simulink library "Lib_Piccolo"  (R2018b)
settings: Solver=VariableStepAuto  StartTime=0.0  StopTime=10.0  RelTol=1e-3
values from neighbouring files (symbols this model uses):
  AccelErrInt2Brakes = 0.15    [SimulationControlConfig16P.m]    (also in SimulationControlConfig16P_LEGACY.m; SimulationControlConfigTAILLESS.m = 0.2; SimulationControlConfigUTAIL.m = 0.2)
  AileronMax = 25    [SimulationControlConfig16P.m]    (also in SimulationControlConfig16P_LEGACY.m; SimulationControlConfigTAILLESS.m; SimulationControlConfigUTAIL.m)
  AileronPower = 0.00268    [SimulationControlConfig16P.m]    (also in SimulationControlConfig16P_LEGACY.m; SimulationControlConfigTAILLESS.m; SimulationControlConfigUTAIL.m)
  AileronSurfaceMax = 45    [SimulationControlConfig16P.m]    (also in SimulationControlConfig16P_LEGACY.m)
  AileronTrim = 0    [SimulationControlConfig16P.m]    (also in SimulationControlConfig16P_LEGACY.m; SimulationControlConfigTAILLESS.m; SimulationControlConfigUTAIL.m)
  Alt = 1000 + TerrainHeight    [SimulationStateConfig.m]
  AltCruise_m = testPlans(testIndx).terrainElevation * 0.3048 + 200    [SimulationControlConfig16P.m]    (also in SimulationControlConfigTAILLESS.m = 1083; SimulationControlConfigUTAIL.m = testPlans(testIndx).terrainElevation * 0.3048 + 152)
  AltitudeRate2PitchCmdIntegratorInit = 0.1    [SimulationControlPre.m]
  AltMax = 10000    [SimulationControlConfig16P.m]    (also in SimulationControlConfig16P_LEGACY.m; SimulationControlConfigTAILLESS.m; SimulationControlConfigUTAIL.m)
  AltMaxAccel = 1.25    [SimulationControlConfig16P.m]    (also in SimulationControlConfig16P_LEGACY.m = 0.9; SimulationControlConfigTAILLESS.m = 1.7; SimulationControlConfigUTAIL.m = 2)
  AltMin = 0    [SimulationControlConfig16P.m]    (also in SimulationControlConfig16P_LEGACY.m; SimulationControlConfigTAILLESS.m; SimulationControlConfigUTAIL.m)
  AltRateCmd2Pitch = 0.50    (= 0.5)    [SimulationControlConfig16P.m]    (also in SimulationControlConfig16P_LEGACY.m = 0.6; SimulationControlConfigTAILLESS.m = 0.2; SimulationControlConfigUTAIL.m = 0.3)
  AltRateError2Pitch = 0.40    (= 0.4)    [SimulationControlConfig16P.m]    (also in SimulationControlConfig16P_LEGACY.m; SimulationControlConfigTAILLESS.m = 0.55; SimulationControlConfigUTAIL.m = 0.55)
  AltRateErrorInt2Pitch = 0.50    (= 0.5)    [SimulationControlConfig16P.m]    (also in SimulationControlConfig16P_LEGACY.m = 0.45; SimulationControlConfigTAILLESS.m; SimulationControlConfigUTAIL.m = 0.75)
  AltRateLpfCutOff = 3    [SimulationControlConfig16P.m]    (also in SimulationControlConfig16P_LEGACY.m; SimulationControlConfigTAILLESS.m = 2; SimulationControlConfigUTAIL.m = 2)
  AutoNosegear2Rudder = 26    [SimulationControlConfig16P.m]    (also in SimulationControlConfig16P_LEGACY.m; SimulationControlConfigTAILLESS.m = 25.2; SimulationControlConfigUTAIL.m = 14)
  b = 5.54    [SimulationControlConfig16P.m]    (also in SimulationControlConfig16P_LEGACY.m; SimulationControlConfigTAILLESS.m = 2.37; SimulationControlConfigUTAIL.m = 2.37)
  Bank2AileronIntegratorInit = 0    [SimulationControlPre.m]
  BankMax_User = BankMax_User/180*pi    (= 0.523598775598)    [SimulationControlConfig16P.m]    (also in SimulationControlConfig16P_LEGACY.m; SimulationControlConfigTAILLESS.m = 0.610865238198; SimulationControlConfigUTAIL.m = 0.628318530718)
  baseLegFlaps = 20    [SimulationControlConfig16P.m]    (also in SimulationControlConfig16P_LEGACY.m = 0; SimulationControlConfigTAILLESS.m = 15; SimulationControlConfigUTAIL.m = 10)
  C = GeneticOpt.C    [SimulationCostFunction.m]
  c = Sw/b    (= 0.841696750903)    [SimulationControlConfig16P.m]    (also in SimulationControlConfig16P_LEGACY.m; SimulationControlConfigTAILLESS.m = 0.354008438819; SimulationControlConfigUTAIL.m = 0.354008438819)
  cell2WheelFactorMG = 5.98    [SimulationSensorConfig16P_LEGACY.m]
  cell2WheelFactorNG = 1    [SimulationSensorConfig16P_LEGACY.m]
  cellSatMaxMG = 15000    [SimulationSensorConfig16P.m]    (also in SimulationSensorConfig16P_LEGACY.m; SimulationSensorConfigTAILLESS7P.m; SimulationSensorConfigUTAIL7P.m)
  cellSatMaxNG = 1000    [SimulationSensorConfig16P.m]    (also in SimulationSensorConfig16P_LEGACY.m; SimulationSensorConfigTAILLESS7P.m; SimulationSensorConfigUTAIL7P.m)
  cellSatMinMG = -15000    [SimulationSensorConfig16P.m]    (also in SimulationSensorConfig16P_LEGACY.m; SimulationSensorConfigTAILLESS7P.m; SimulationSensorConfigUTAIL7P.m)
  cellSatMinNG = -1000    [SimulationSensorConfig16P.m]    (also in SimulationSensorConfig16P_LEGACY.m; SimulationSensorConfigTAILLESS7P.m; SimulationSensorConfigUTAIL7P.m)
  CL_Limit = CL_Max    (= 0.54)    [SimulationControlConfig16P.m]    (also in SimulationControlConfig16P_LEGACY.m; SimulationControlConfigTAILLESS.m; SimulationControlConfigUTAIL.m = 0.53)
  CL_Max = 0.54    [SimulationControlConfig16P.m]    (also in SimulationControlConfig16P_LEGACY.m; SimulationControlConfigTAILLESS.m; SimulationControlConfigUTAIL.m = 0.53)
  CL_Max_Nom = 0.465    [SimulationControlConfig16P.m]    (also in SimulationControlConfig16P_LEGACY.m; SimulationControlConfigTAILLESS.m = 0.39; SimulationControlConfigUTAIL.m)
  CL_Min = 0    [SimulationControlConfig16P.m]    (also in SimulationControlConfig16P_LEGACY.m; SimulationControlConfigTAILLESS.m; SimulationControlConfigUTAIL.m)
  ClimbMaxFraction = 0.35    [SimulationControlConfig16P.m]    (also in SimulationControlConfig16P_LEGACY.m = 0.24; SimulationControlConfigTAILLESS.m = 0.19; SimulationControlConfigUTAIL.m = 0.21)
  ClimboutMaxBank = 7.0    (= 7)    [SimulationControlConfig16P.m]    (also in SimulationControlConfig16P_LEGACY.m; SimulationControlConfigTAILLESS.m = 5; SimulationControlConfigUTAIL.m)
  ClimboutTimer = 7.0    (= 7)    [SimulationControlConfig16P.m]    (also in SimulationControlConfig16P_LEGACY.m; SimulationControlConfigTAILLESS.m; SimulationControlConfigUTAIL.m)
  dCl_per_dFlap = 0.005581818    [SimulationControlConfig16P.m]    (also in SimulationControlConfig16P_LEGACY.m = 0; SimulationControlConfigTAILLESS.m = 0; SimulationControlConfigUTAIL.m = 0)
  DecelerationCmd = 3.1    [SimulationControlConfig16P.m]    (also in SimulationControlConfig16P_LEGACY.m; SimulationControlConfigTAILLESS.m = 0.1; SimulationControlConfigUTAIL.m = 0.1)
  DeRotateLogicEndTimer = abs((NoseDownLimit_Deg-1)/DeRotateRamp_Dps)    [SimulationControlConfig16P.m]    (also in SimulationControlConfig16P_LEGACY.m; SimulationControlConfigTAILLESS.m; SimulationControlConfigUTAIL.m)
  DeRotateLogicHoldNoseUpTimer = 0.1    [SimulationControlConfig16P.m]    (also in SimulationControlConfig16P_LEGACY.m; SimulationControlConfigTAILLESS.m; SimulationControlConfigUTAIL.m)
  DeRotateLogicTimerTimeout = 2    [SimulationControlConfig16P.m]    (also in SimulationControlConfig16P_LEGACY.m; SimulationControlConfigTAILLESS.m; SimulationControlConfigUTAIL.m)
  DeRotateLowerCmdSaturation = 0    [SimulationControlConfig16P.m]    (also in SimulationControlConfig16P_LEGACY.m; SimulationControlConfigTAILLESS.m; SimulationControlConfigUTAIL.m)
  DeRotateRamp_Dps = 3    [SimulationControlConfig16P.m]    (also in SimulationControlConfig16P_LEGACY.m; SimulationControlConfigTAILLESS.m = 8; SimulationControlConfigUTAIL.m = 8)
  DeRotateUpperCmdSaturation = 7    [SimulationControlConfig16P.m]    (also in SimulationControlConfig16P_LEGACY.m; SimulationControlConfigTAILLESS.m; SimulationControlConfigUTAIL.m)
  DescentMaxFraction = 0.22    [SimulationControlConfig16P.m]    (also in SimulationControlConfig16P_LEGACY.m = 0.2; SimulationControlConfigTAILLESS.m = 0.17; SimulationControlConfigUTAIL.m = 0.17)
  DesktopSimTerrainOffset_m = 0.406    [SimulationAircraftConfig.m]
  downwindFlaps = 0    [SimulationControlConfig16P.m]    (also in SimulationControlConfig16P_LEGACY.m; SimulationControlConfigTAILLESS.m; SimulationControlConfigUTAIL.m)
  DP_init = 0.5*1.225*V_init^2    [SimulationControlConfig16P.m]    (also in SimulationControlConfig16P_LEGACY.m; SimulationControlConfigTAILLESS.m; SimulationControlConfigUTAIL.m)
  dscNoiseMG = 1    [SimulationSensorConfig16P_LEGACY.m]
  dscNoiseNG = 0.25    [SimulationSensorConfig16P_LEGACY.m]
  DSCnumBits = 24    [SimulationSensorConfig16P.m]    (also in SimulationSensorConfig16P_LEGACY.m; SimulationSensorConfigTAILLESS7P.m; SimulationSensorConfigUTAIL7P.m)
  DSCRangeMaxMG = 15000    [SimulationSensorConfig16P.m]    (also in SimulationSensorConfig16P_LEGACY.m; SimulationSensorConfigTAILLESS7P.m; SimulationSensorConfigUTAIL7P.m)
  DSCRangeMaxNG = 1000    [SimulationSensorConfig16P.m]    (also in SimulationSensorConfig16P_LEGACY.m; SimulationSensorConfigTAILLESS7P.m; SimulationSensorConfigUTAIL7P.m)
  DSCRangeMinMG = -15000    [SimulationSensorConfig16P.m]    (also in SimulationSensorConfig16P_LEGACY.m; SimulationSensorConfigTAILLESS7P.m; SimulationSensorConfigUTAIL7P.m)
  DSCRangeMinNG = -1000    [SimulationSensorConfig16P.m]    (also in SimulationSensorConfig16P_LEGACY.m; SimulationSensorConfigTAILLESS7P.m; SimulationSensorConfigUTAIL7P.m)
  dt = DLLSim.dt    [SimulationTimeStep.m]    (also in SimulationTrim.m = 0.02)
  EarlyTouchdownThreshold = 3.0    (= 3)    [SimulationControlConfig16P.m]    (also in SimulationControlConfig16P_LEGACY.m; SimulationControlConfigTAILLESS.m = 2.2; SimulationControlConfigUTAIL.m = 2.5)
  ElevatorDeflectionRate = 15    [SimulationControlConfig16P.m]    (also in SimulationControlConfig16P_LEGACY.m = 12; SimulationControlConfigTAILLESS.m = 10; SimulationControlConfigUTAIL.m = 12)
  ElevatorMax = 25    [SimulationControlConfig16P.m]    (also in SimulationControlConfig16P_LEGACY.m; SimulationControlConfigTAILLESS.m; SimulationControlConfigUTAIL.m)
  ElevatorPower = -0.002209    [SimulationControlConfig16P.m]    (also in SimulationControlConfig16P_LEGACY.m; SimulationControlConfigTAILLESS.m = -0.002956; SimulationControlConfigUTAIL.m = -0.00205983)
  ElevatorTrim = -3.5    [SimulationControlConfig16P.m]    (also in SimulationControlConfig16P_LEGACY.m; SimulationControlConfigTAILLESS.m = -6; SimulationControlConfigUTAIL.m = -8)
  elevonBias = 0    [SimulationControlConfig16P.m]    (also in SimulationControlConfig16P_LEGACY.m; SimulationControlConfigTAILLESS.m; SimulationControlConfigUTAIL.m)
  Enable_TAS_Protection = 0    [SimulationControlConfig16P.m]    (also in SimulationControlConfig16P_LEGACY.m; SimulationControlConfigTAILLESS.m; SimulationControlConfigUTAIL.m)
  EnableCrossTrackAbort = 1    [SimulationControlConfig16P.m]    (also in SimulationControlConfigTAILLESS.m; SimulationControlConfigUTAIL.m)
  EnergyBandwidth = 0.02    [SimulationControlConfig16P.m]    (also in SimulationControlConfig16P_LEGACY.m; SimulationControlConfigTAILLESS.m = 0.06; SimulationControlConfigUTAIL.m = 0.06)
  EngineLhFuelCut = 0    [SimulationAircraftConfig.m]
  EngineRhFuelCut = 0    [SimulationAircraftConfig.m]
  FastThrottleRate = 0.075    [SimulationControlConfig16P.m]    (also in SimulationControlConfig16P_LEGACY.m = 0.05; SimulationControlConfigTAILLESS.m = 0.1; SimulationControlConfigUTAIL.m = 0.1)
  FilterWarmUpTime = 2    [SimulationSensorConfig16P.m]    (also in SimulationSensorConfig16P_LEGACY.m; SimulationSensorConfigTAILLESS7P.m; SimulationSensorConfigUTAIL7P.m)
  finalApproachFlaps = 20    [SimulationControlConfig16P.m]    (also in SimulationControlConfig16P_LEGACY.m = 0; SimulationControlConfigTAILLESS.m = 22; SimulationControlConfigUTAIL.m = 10)
  FinalDescentSlope_Deg = testPlans(testIndx).descentSlope    [SimulationControlConfig16P.m]    (also in SimulationControlConfig16P_LEGACY.m; SimulationControlConfigTAILLESS.m; SimulationControlConfigUTAIL.m)
  flapMax = 0    [SimulationControlConfig16P.m]    (also in SimulationControlConfig16P_LEGACY.m; SimulationControlConfigTAILLESS.m; SimulationControlConfigUTAIL.m)
  flapRate = 7.5    [SimulationControlConfig16P.m]    (also in SimulationControlConfig16P_LEGACY.m; SimulationControlConfigTAILLESS.m = 6.6; SimulationControlConfigUTAIL.m)
  FlareHeight = 5    [SimulationControlConfig16P.m]    (also in SimulationControlConfig16P_LEGACY.m = 4.8; SimulationControlConfigTAILLESS.m = 2.5; SimulationControlConfigUTAIL.m = 2)
  FlareVerticalRate_mps = -0.4    [SimulationControlConfig16P.m]    (also in SimulationControlConfig16P_LEGACY.m = -0.5; SimulationControlConfigTAILLESS.m = -0.15; SimulationControlConfigUTAIL.m = -0.15)
  Fp_Aileron = 0.55*2*pi*RollRateLpfCutoff*dt    [SimulationControlConfig16P.m]    (also in SimulationControlConfig16P_LEGACY.m; SimulationControlConfigTAILLESS.m; SimulationControlConfigUTAIL.m)
  Fp_Alt = 0.55*AltBandwidth    (= 0.099)    [SimulationControlConfig16P.m]    (also in SimulationControlConfig16P_LEGACY.m; SimulationControlConfigTAILLESS.m = 0.587477826221; SimulationControlConfigUTAIL.m = 0.69115038379)
  Fp_AltRate = 0.55*2*pi*AltRateLpfCutOff*dt    [SimulationControlConfig16P.m]    (also in SimulationControlConfig16P_LEGACY.m; SimulationControlConfigTAILLESS.m; SimulationControlConfigUTAIL.m)
  Fp_Elevator = 0.55*2*pi*PitchRateLpfCutoff*dt    [SimulationControlConfig16P.m]    (also in SimulationControlConfig16P_LEGACY.m; SimulationControlConfigTAILLESS.m; SimulationControlConfigUTAIL.m)
  Fp_Energy = 0.55*2*pi*EnergyBandwidth    (= 0.069115038379)    [SimulationControlConfig16P.m]    (also in SimulationControlConfig16P_LEGACY.m; SimulationControlConfigTAILLESS.m = 0.207345115137; SimulationControlConfigUTAIL.m = 0.207345115137)
  Fp_Energy2 = 0.55*2*pi*EnergyBandwidth*dt    [SimulationControlConfig16P.m]    (also in SimulationControlConfig16P_LEGACY.m; SimulationControlConfigTAILLESS.m; SimulationControlConfigUTAIL.m)
  Fp_Pitch = 0.55*2*pi*PitchBandwidth    (= 2.76460153516)    [SimulationControlConfig16P.m]    (also in SimulationControlConfig16P_LEGACY.m = 3.11017672705; SimulationControlConfigTAILLESS.m = 3.80132711084; SimulationControlConfigUTAIL.m = 2.41902634326)
  Fp_Pitch_2 = 0.55*2*pi*PitchBandwidth*dt    [SimulationControlConfig16P.m]    (also in SimulationControlConfig16P_LEGACY.m; SimulationControlConfigTAILLESS.m; SimulationControlConfigUTAIL.m)
  Fp_Roll = RollBandwidth^2    (= 1)    [SimulationControlConfig16P.m]    (also in SimulationControlConfig16P_LEGACY.m = 1.44; SimulationControlConfigTAILLESS.m; SimulationControlConfigUTAIL.m)
  Fp_Rudder = 0.55*2*pi*YawRateLpfCutoff*dt    [SimulationControlConfig16P.m]    (also in SimulationControlConfig16P_LEGACY.m; SimulationControlConfigTAILLESS.m; SimulationControlConfigUTAIL.m)
  Fp_TAS = 0.55*2*pi*TASBandwidth    (= 0.103672557568)    [SimulationControlConfig16P.m]    (also in SimulationControlConfig16P_LEGACY.m; SimulationControlConfigTAILLESS.m = 0.172787595947; SimulationControlConfigUTAIL.m = 0.172787595947)
  Fp_TAS_Filter = 2*pi*TasLpfCutoff*dt    [SimulationControlConfig16P.m]    (also in SimulationControlConfig16P_LEGACY.m; SimulationControlConfigTAILLESS.m; SimulationControlConfigUTAIL.m)
  Fp_Turn = 0.55*2*pi*TurnErrLPFcutoff    (= 0.0345575191895)    [SimulationControlConfig16P.m]    (also in SimulationControlConfig16P_LEGACY.m; SimulationControlConfigTAILLESS.m = 0.172787595947; SimulationControlConfigUTAIL.m = 0.172787595947)
  Fp_TurnDerr = 0.55*2*pi*TurnDerivativeLPFcutoff    (= 0.0345575191895)    [SimulationControlConfig16P.m]    (also in SimulationControlConfig16P_LEGACY.m; SimulationControlConfigTAILLESS.m = 0.172787595947; SimulationControlConfigUTAIL.m = 0.172787595947)
  FTV = 3    [SimulationAircraftConfig.m]
  ftvStaticPositionError = 1/1.18    (= 0.847457627119)    [SimulationSensorConfig16P.m]    (also in SimulationSensorConfig16P_LEGACY.m; SimulationSensorConfigTAILLESS7P.m = 1; SimulationSensorConfigUTAIL7P.m = 1)
  g = 9.81    [SimulationStateConfig.m]
  GustSpd_Kts = testPlans(testIndx).gustSpd    [SimulationStateConfig.m]
  GustTriggerVal = testPlans(testIndx).gustTriggerVal    [SimulationStateConfig.m]
  HeadingErr2TurnRate = 0.5    [SimulationControlConfig16P.m]    (also in SimulationControlConfig16P_LEGACY.m; SimulationControlConfigTAILLESS.m; SimulationControlConfigUTAIL.m)
  HeadingErrDer2TurnRate = 0.3    [SimulationControlConfig16P.m]    (also in SimulationControlConfig16P_LEGACY.m; SimulationControlConfigTAILLESS.m; SimulationControlConfigUTAIL.m)
  IASbounce = IASstall*0.8    [SimulationControlPre.m]
  IAScruiseCMD = sqrt(2*m*9.81/(1.225*Sw*CL_cruise))    [SimulationControlConfig16P.m]    (also in SimulationControlConfig16P_LEGACY.m; SimulationControlConfigTAILLESS.m; SimulationControlConfigUTAIL.m)
  IASfinalCMD = 1.12 * IASmin    [SimulationControlConfig16P.m]    (also in SimulationControlConfig16P_LEGACY.m = 1.10 * IASmin; SimulationControlConfigTAILLESS.m = 1.10 * IASmin; SimulationControlConfigUTAIL.m = 1.15 * IASmin)
  IASflareCMD = IASstall    [SimulationControlConfig16P.m]    (also in SimulationControlConfig16P_LEGACY.m; SimulationControlConfigTAILLESS.m; SimulationControlConfigUTAIL.m)
  IASmax = 64    [SimulationControlConfig16P.m]    (also in SimulationControlConfig16P_LEGACY.m = 46; SimulationControlConfigTAILLESS.m = 38.58; SimulationControlConfigUTAIL.m = 35)
  IASmin = sqrt(2*m*9.81/(1.225*Sw*0.9*CL_Max_Nom))    [SimulationControlConfig16P.m]    (also in SimulationControlConfig16P_LEGACY.m; SimulationControlConfigTAILLESS.m; SimulationControlConfigUTAIL.m)
  IASshortCMD = IASstall    [SimulationControlConfig16P.m]    (also in SimulationControlConfig16P_LEGACY.m; SimulationControlConfigTAILLESS.m; SimulationControlConfigUTAIL.m)
  IASstall = sqrt(2*m*9.81/(1.225*Sw*CL_Max))    [SimulationControlConfig16P.m]    (also in SimulationControlConfig16P_LEGACY.m; SimulationControlConfigTAILLESS.m; SimulationControlConfigUTAIL.m)
  inFlight = 1    [SimulationControlConfig16P.m]    (also in SimulationControlConfigTAILLESS.m; SimulationControlConfigUTAIL.m)
  JetCatOffset = 5    [SimulationControlConfig16P.m]    (also in SimulationControlConfig16P_LEGACY.m)
  LaunchRollingElevator = -1.5    [SimulationControlConfig16P.m]    (also in SimulationControlConfig16P_LEGACY.m; SimulationControlConfigTAILLESS.m = 1; SimulationControlConfigUTAIL.m = 1)
  ldg_NosegearMax = 10    [SimulationControlConfig16P.m]    (also in SimulationControlConfig16P_LEGACY.m; SimulationControlConfigTAILLESS.m; SimulationControlConfigUTAIL.m)
  ldg_TrackVyErrInt2Nosegear = 0.1250    (= 0.125)    [SimulationControlConfig16P.m]    (also in SimulationControlConfig16P_LEGACY.m; SimulationControlConfigTAILLESS.m = 0.00714285714286; SimulationControlConfigUTAIL.m = 0.00714285714286)
  ldg_TrackVyErrPro2Nosegear = 0.35    [SimulationControlConfig16P.m]    (also in SimulationControlConfig16P_LEGACY.m; SimulationControlConfigTAILLESS.m = 0.0546666666667; SimulationControlConfigUTAIL.m = 0.0546666666667)
  ldg_TrackY2Vy = 0.07    [SimulationControlConfig16P.m]    (also in SimulationControlConfig16P_LEGACY.m; SimulationControlConfigTAILLESS.m = 0.17; SimulationControlConfigUTAIL.m = 0.17)
  ldg_Vy2NosegearScalingPower = 1.075    [SimulationControlConfig16P.m]    (also in SimulationControlConfig16P_LEGACY.m; SimulationControlConfigTAILLESS.m = 0.6; SimulationControlConfigUTAIL.m = 0.5)
  ldg_Y2VyScalingPower = 0.175    [SimulationControlConfig16P.m]    (also in SimulationControlConfig16P_LEGACY.m; SimulationControlConfigTAILLESS.m = 0; SimulationControlConfigUTAIL.m = 0)
  ldg_YawRate2Nosegear = 0.175    [SimulationControlConfig16P.m]    (also in SimulationControlConfig16P_LEGACY.m; SimulationControlConfigTAILLESS.m = 0.065; SimulationControlConfigUTAIL.m = 0.065)
  LiftSlope = 0.064285    [SimulationControlConfig16P.m]    (also in SimulationControlConfig16P_LEGACY.m; SimulationControlConfigTAILLESS.m = 0.058631; SimulationControlConfigUTAIL.m)
  LPFaileronInit = 0    [SimulationControlPre.m]
  LPFclestInit = 0    [SimulationControlPre.m]
  LPFenergyFFInit = 0    [SimulationControlPre.m]
  LPFtasInit = V_init + 2    [SimulationControlPre.m]
  LPFthrottleInit = ThrottleTrim    [SimulationControlPre.m]
  LPFturnErrInit = 0    [SimulationControlPre.m]
  ... (+115 more)
undefined symbols (not defined in the file or in its folder): abortFlag, alphaHPF, apmDelay, BRWNOUT, CRAWOR, CRAWUR, DiscIntNeverNeededParam, DLLSim, DLLSimStep, ECOMOR, ECOMUR, Fp_Tas, GustTrigger_HeightAgl_m, IPSTAT, LCINTEG, Ldg_Persist_Time, LOWER_FLAGS, MSG_ENABLE, NoiseStd, OLDVAL, OVERRIDE_ENABLE, OVERRIDE_VALUE, REBOOT, reversionEnable, revIASMax, revIASMin, revPitchMax, revPitchMin, revPitchRateMax, revRollMax, revRollRateMax, SAMPLE, SCALON, SensorModel, sigbuilder_block, Sim_Vx, Sim_Vy, Sim_Vz, Sim_Xpos, Sim_Ypos, Sim_Zpos, SYSOR, SYSUR, TARE, TEMPOR, TEMPUR, testIndx, testPlan, testPlans, Trim_piccoloInCmd, Trim_REFSI_FD_IN_nmodeCgShifterCmd_Ft, Trim_REFSI_FD_IN_nmodeFlapLhIBCmd_Deg, Trim_REFSI_FD_IN_nmodeFlapLhOBCmd_Deg, Trim_REFSI_FD_IN_nmodeFlapRhIBCmd_Deg, Trim_REFSI_FD_IN_nmodeFlapRhOBCmd_Deg, Trim_REFSI_FD_IN_nmodeSlatLhCmd_Deg, Trim_REFSI_FD_IN_nmodeSlatRhCmd_Deg, Trim_REFSI_FD_IN_nmodeSplrLhInbdCmd_Deg, Trim_REFSI_FD_IN_nmodeSplrLhOutbdCmd_Deg ... (+5)
libraries: simulink x866, aerolibconvert2 x60, $bdroot x52, aerolibatmos2 x5, dspswit3 x5, simulink_extras x4, dsparch4 x2, Lib_Piccolo_Alt x2, eeGeneralControl x1, dspindex x1
(part 28 of 44)

== system Lib_Piccolo/Ground Detection Systems/WoW Wrapper/Variant Subsystem/Load Cell WoW Model 18 ==
  note: Scaling relationship between measured load cell load and WoW load excluded since loads provided from FDM are already at wheel
  note: CANOpen transport delay from DSC to K2 is <1ms. Addtional delay here also accounts for worst case asynchronicity between DSC PDO and K2 sampling. Load phase delay defined in workspace.
  note: Data Formatting for Piccolo Communications
  note: K2 Data Acquisition and Processing
  note: These signals are sent on the CMD and TELEM CAN Bus in the 0x3280000 ID Message
  note: Inputs to WOW block are 32-bit float (IEEE 754) direct from DSC with appropriate cell scaling applied. Re-encoded integer loads are only used for telemetry output.
  note: Load Cell Model
  note: DSC Model
  Piccolo_AP_Mode : Inport
  Bus Element In5 : Inport  Port=2  PortName=WoW_Bus_In  Element=ZgrndRhLbs
  Bus Element In4 : Inport  Port=2  PortName=WoW_Bus_In  Element=ZgrndLhLbs
  Bus Element In1 : Inport  Port=2  PortName=WoW_Bus_In  Element=ZgrndNgLbs
  Bus Creator : BusCreator  Inputs=2
  Bus Creator1 : BusCreator  Inputs=3
  Cell to Wheel Load MGL : Gain
  Cell to Wheel Load MGR : Gain
  Cell to Wheel Load NG : Gain
  Conversion - MGL : $bdroot/Ground Detection Systems/WoW Wrapper/Variant Subsystem/Load Cell WoW Model 18/Conversion - NG  SystemSampleTime=-1  Latency=0  AutoFrameSizeCalculation=off
  Conversion - MGR : $bdroot/Ground Detection Systems/WoW Wrapper/Variant Subsystem/Load Cell WoW Model 18/Conversion - NG  SystemSampleTime=-1  Latency=0  AutoFrameSizeCalculation=off
  Conversion - NG : Subsystem
  DSC Noise L : RandomNumber  Variance=(SensorModel.WOW.Cell.dscNoiseMG/6)^2  Seed=20  SampleTime=dt
  DSC Noise N : RandomNumber  Variance=(SensorModel.WOW.Cell.dscNoiseNG/6)^2  Seed=10  SampleTime=dt
  DSC Noise R : RandomNumber  Variance=(SensorModel.WOW.Cell.dscNoiseMG/6)^2  Seed=30  SampleTime=dt
  Data Type Conversion : DataTypeConversion
  Data Type Conversion1 : DataTypeConversion
  Data Type L : DataTypeConversion  OutDataTypeStr=single
  Data Type N : DataTypeConversion  OutDataTypeStr=single
  Data Type R : DataTypeConversion  OutDataTypeStr=single
  Delay1 : Delay  DelayLength=SensorModel.WOW.Cell.WOWtransportDelay
  Delay2 : Delay  DelayLength=SensorModel.WOW.Cell.WOWtransportDelay
  Delay3 : Delay  DelayLength=SensorModel.WOW.Cell.WOWtransportDelay
  Gain : Gain  Gain=100
  Ground : Ground
  MGL_DSC_FAIL_INPUT : Constant  Value=SensorModel.WOW.Cell.MGL_FAIL  OutDataTypeStr=uint8
  MGR_DSC_FAIL_INPUT : Constant  Value=SensorModel.WOW.Cell.MGR_FAIL  OutDataTypeStr=uint8
  Quantization L : Quantizer  QuantizationInterval=(SensorModel.WOW.Cell.calibrationSlopeMG * (SensorModel.WOW.Cell.fullScaleRange/SensorModel.WOW.Cell.effectiveCounts)) / SensorModel.WOW.Cell.cell2WheelFactorMG
  Quantization N : Quantizer  QuantizationInterval=(SensorModel.WOW.Cell.calibrationSlopeNG * (SensorModel.WOW.Cell.fullScaleRange/SensorModel.WOW.Cell.effectiveCounts)) / SensorModel.WOW.Cell.cell2WheelFactorNG
  Quantization R : Quantizer  QuantizationInterval=(SensorModel.WOW.Cell.calibrationSlopeMG * (SensorModel.WOW.Cell.fullScaleRange/SensorModel.WOW.Cell.effectiveCounts)) / SensorModel.WOW.Cell.cell2WheelFactorMG
  Re-Encoding L : Quantizer  QuantizationInterval=(SensorModel.WOW.Cell.satMaxMG-SensorModel.WOW.Cell.satMinMG)/(2^SensorModel.WOW.Cell.numBits)
  Re-Encoding N : Quantizer  QuantizationInterval=(SensorModel.WOW.Cell.satMaxNG-SensorModel.WOW.Cell.satMinNG)/(2^SensorModel.WOW.Cell.numBits)
  Re-Encoding R : Quantizer  QuantizationInterval=(SensorModel.WOW.Cell.satMaxMG-SensorModel.WOW.Cell.satMinMG)/(2^SensorModel.WOW.Cell.numBits)  LinearizeAsGain=off
  Signal Specification L : SignalSpecification  OutDataTypeStr=single  Dimensions=[1 1]  SampleTime=dt
  Signal Specification N : SignalSpecification  OutDataTypeStr=single  Dimensions=[1 1]  SampleTime=dt
  Signal Specification R : SignalSpecification  OutDataTypeStr=single  Dimensions=[1 1]  SampleTime=dt
  Software Saturation L : Saturate  UpperLimit=SensorModel.WOW.Cell.satMaxMG  LowerLimit=SensorModel.WOW.Cell.satMinMG
  Software Saturation N : Saturate  UpperLimit=SensorModel.WOW.Cell.satMaxNG  LowerLimit=SensorModel.WOW.Cell.satMinNG
  Software Saturation R : Saturate  UpperLimit=SensorModel.WOW.Cell.satMaxMG  LowerLimit=SensorModel.WOW.Cell.satMinMG
  Subsystem : Subsystem
  Sum : Sum  Inputs=|++
  Sum1 : Sum  Inputs=|++
  Sum2 : Sum  Inputs=|++
  Terminator : Terminator
  Wheel to Cell Load MGL : Gain  Gain=SensorModel.WOW.Cell.cell2WheelFactorMG
  Wheel to Cell Load MGR : Gain  Gain=SensorModel.WOW.Cell.cell2WheelFactorMG
  Wheel to Cell Load NG : Gain  Gain=SensorModel.WOW.Cell.cell2WheelFactorNG
  WOW_Bus_Out : Outport
  tag scope: Sim_WOW_L_N=global, Sim_WOW_Logic_Disable=global, Sim_WOW_NG_N=global, Sim_WOW_R_N=global
  wires:
  Subsystem/3(WOW_Filt_MGR_N) -> [Sim_WOW_R_N]
  Subsystem/2(WOW_Filt_MGL_N) -> [Sim_WOW_L_N]
  Subsystem/1(WOW_Filt_NG_N) -> [Sim_WOW_NG_N]
  Piccolo_AP_Mode/1 -> Subsystem/5(PICCOLO_AP_MODE)
  Cell to Wheel Load MGR/1 -> Subsystem/3(WOW_MGR_N)  "Sim.WOW_R_N"
  Ground/1 -> Subsystem/4(RESET)
  Cell to Wheel Load MGL/1 -> Subsystem/2(WOW_MGL_N)  "Sim.WOW_L_N"
  Cell to Wheel Load NG/1 -> Subsystem/1(WOW_NG_N)  "Sim.WOW_NG_N"
  Subsystem/4(Contact) -> Data Type Conversion/1, Gain/1
  Bus Creator/1 -> WOW_Bus_Out/1
  Data Type Conversion/1 -> Bus Creator/1  "ContactBool"
  Gain/1 -> Data Type Conversion1/1
  Data Type Conversion1/1 -> Bus Creator/2  "WoWPcnt"
  Signal Specification L/1 -> Software Saturation L/1
  Software Saturation L/1 -> Cell to Wheel Load MGL/1, Re-Encoding L/1
  Signal Specification R/1 -> Software Saturation R/1
  Software Saturation R/1 -> Cell to Wheel Load MGR/1, Re-Encoding R/1
  Re-Encoding L/1 -> Wheel to Cell Load MGL/1
  Re-Encoding R/1 -> Wheel to Cell Load MGR/1
  Signal Specification N/1 -> Software Saturation N/1
  Software Saturation N/1 -> Cell to Wheel Load NG/1, Re-Encoding N/1
  Re-Encoding N/1 -> Wheel to Cell Load NG/1
  Wheel to Cell Load MGR/1 -> Bus Creator1/3  "Sim.328_MGR_Cell_Telem_N"
  Wheel to Cell Load MGL/1 -> Bus Creator1/2  "Sim.328_MGL_Cell_Telem_N"
  Wheel to Cell Load NG/1 -> Bus Creator1/1  "Sim.328_NG_Cell_Telem_N"
  Bus Creator1/1 -> Terminator/1  "Sim.328_Integer_Loads"
  MGL_DSC_FAIL_INPUT/1 -> Subsystem/7(MGL_DSC_FAIL)
  MGR_DSC_FAIL_INPUT/1 -> Subsystem/6(MGR_DSC_FAIL)
  Subsystem/5(WOW_Logic_Disable) -> [Sim_WOW_Logic_Disable]
  DSC Noise L/1 -> Sum/2
  Conversion - MGL/1 -> Sum/1
  Conversion - NG/1(N) -> Sum2/1
  Conversion - MGR/1 -> Sum1/1
  DSC Noise N/1 -> Sum2/2
  Sum/1 -> Quantization L/1
  Bus Element In1/1 -> Conversion - NG/1(Lbf)
  Delay1/1 -> Signal Specification L/1
  Sum1/1 -> Quantization R/1
  Sum2/1 -> Quantization N/1
  Quantization N/1 -> Data Type N/1
  Quantization L/1 -> Data Type L/1
  Delay2/1 -> Signal Specification R/1
  Data Type R/1 -> Delay2/1
  Bus Element In5/1 -> Conversion - MGR/1
  Quantization R/1 -> Data Type R/1
  Data Type N/1 -> Delay3/1
  Data Type L/1 -> Delay1/1
  Delay3/1 -> Signal Specification N/1
  DSC Noise R/1 -> Sum1/2
  Bus Element In4/1 -> Conversion - MGL/1

== system Lib_Piccolo/Ground Detection Systems/WoW Wrapper/Variant Subsystem/Load Cell WoW Model 20 ==
  note: K2 System Boundary
  note: Wheel loads from FDM, units of lbf .
  note: CANOpen transport delay from DSC to K2 is <1ms. Addtional delay here also accounts for worst case asynchronicity between DSC PDO and K2 sampling. Load phase delay defined in workspace.
  note: Data Formatting for Piccolo Communications
  note: K2 Data Acquisition and Processing
  note: DSC Model
  note: Load Cell Model
  note: These signals are sent on the CMD and TELEM CAN Bus in the 0x3280000 ID Message
  note: This subsystem is auto-coded to generate the WOW class as integrated by K2. Inports and Outports defined here will constitute the class interface.
  note: Calibrated/converted Wheel loads, as used by WOW logic, units of N .
      |
      | This subsystem is auto-coded and implements signal conditioning of loads prior to use in WOW logic. Inports and Outports defined here will constitute the class interface.
  note: Converted to Cell loads, units of N .
  note: Quantized DSC loads, units of N .
  Piccolo_AP_Mode : Inport
  Bus Element In5 : Inport  Port=2  PortName=WoW_Bus_In  Element=ZgrndRhLbs
  Bus Element In4 : Inport  Port=2  PortName=WoW_Bus_In  Element=ZgrndLhLbs
  Bus Element In1 : Inport  Port=2  PortName=WoW_Bus_In  Element=ZgrndNgLbs
  Bus Creator : BusCreator  Inputs=2
  Bus Selector : BusSelector  OutputSignals=CONTACT
  Bus Formatting MGL : Subsystem
  Bus Formatting MGR : Subsystem
  Bus Formatting NG : Subsystem
  Constant1 : Constant  Value=0  OutDataTypeStr=boolean
  Constant3 : Constant  Value=0  OutDataTypeStr=boolean
  DSC Data Acquisition : Subsystem
  DSC Load Conversion : $bdroot/DSC Load Conversion  SystemSampleTime=-1
  Data Type Conversion : DataTypeConversion
  Data Type Conversion1 : DataTypeConversion
  Data Type Conversion2 : DataTypeConversion  OutDataTypeStr=uint8
  Delay1 : Delay  DelayLength=SensorModel.WOW.Cell.WOWtransportDelay
  Delay2 : Delay  DelayLength=SensorModel.WOW.Cell.WOWtransportDelay
  Delay3 : Delay  DelayLength=SensorModel.WOW.Cell.WOWtransportDelay
  Gain : Gain  Gain=100
  Load Cell and Unit Conversion : Subsystem
  Re-Encoding L : Quantizer  QuantizationInterval=(SensorModel.WOW.Cell.satMaxMG-SensorModel.WOW.Cell.satMinMG)/(2^SensorModel.WOW.Cell.numBits)
  Re-Encoding N : Quantizer  QuantizationInterval=(SensorModel.WOW.Cell.satMaxNG-SensorModel.WOW.Cell.satMinNG)/(2^SensorModel.WOW.Cell.numBits)
  Re-Encoding R : Quantizer  QuantizationInterval=(SensorModel.WOW.Cell.satMaxMG-SensorModel.WOW.Cell.satMinMG)/(2^SensorModel.WOW.Cell.numBits)  LinearizeAsGain=off
  Saturation L : Saturate  UpperLimit=SensorModel.WOW.Cell.satMaxMG  LowerLimit=SensorModel.WOW.Cell.satMinMG
  Saturation N : Saturate  UpperLimit=SensorModel.WOW.Cell.satMaxNG  LowerLimit=SensorModel.WOW.Cell.satMinNG
  Saturation R : Saturate  UpperLimit=SensorModel.WOW.Cell.satMaxMG  LowerLimit=SensorModel.WOW.Cell.satMinMG
  Signal Specification L : SignalSpecification  OutDataTypeStr=single  Dimensions=[1 1]  SampleTime=dt
  Signal Specification N : SignalSpecification  OutDataTypeStr=single  Dimensions=[1 1]  SampleTime=dt
  Signal Specification R : SignalSpecification  OutDataTypeStr=single  Dimensions=[1 1]  SampleTime=dt
  Subsystem : Subsystem
  Terminator{,1..10} (11 alike) : Terminator
  WOW Module : Subsystem
  WOW_Bus_Out : Outport
  tag scope: Sim_WOW_Output_Disable=global
  wires:
  Piccolo_AP_Mode/1 -> WOW Module/1(PICCOLO_AP_MODE)
  Signal Specification R/1 -> Saturation R/1, DSC Load Conversion/3  "Sim.MGR_DSC_Load_N"
  Signal Specification L/1 -> Saturation L/1, DSC Load Conversion/2  "Sim.MGL_DSC_Load_N"
  Signal Specification N/1 -> DSC Load Conversion/1, Saturation N/1  "Sim.NG_DSC_Load_N"
  Bus Selector/1 -> Data Type Conversion2/1  "<CONTACT>"
  Bus Creator/1 -> WOW_Bus_Out/1
  Data Type Conversion/1 -> Bus Creator/1  "ContactBool"
  Gain/1 -> Data Type Conversion1/1
  Data Type Conversion1/1 -> Bus Creator/2  "WoWPcnt"
  Delay1/1 -> Signal Specification L/1
  Delay2/1 -> Signal Specification R/1
  Delay3/1 -> Signal Specification N/1
  Re-Encoding R/1 -> Terminator10/1  "Sim.328_MGR_DSC_Load_N"
  Re-Encoding L/1 -> Terminator9/1  "Sim.328_MGL_DSC_Load_N"
  Re-Encoding N/1 -> Terminator/1  "Sim.328_NG_DSC_Load_N"
  WOW Module/2(WOW_OUTPUT_DISABLE) -> [Sim_WOW_Output_Disable]
  Data Type Conversion2/1 -> Gain/1, Data Type Conversion/1
  Constant3/1 -> WOW Module/2(NRC_ACTIVE)
  Constant1/1 -> WOW Module/6(INITIALIZE)
  Subsystem/1(User Cmds) -> WOW Module/7(User_Cmd_In)
  WOW Module/1(Detection) -> Bus Selector/1
  WOW Module/3(NG_Out) -> Terminator1/1
  WOW Module/5(MGR_Out) -> Terminator2/1
  WOW Module/4(MGL_Out) -> Terminator3/1
  WOW Module/6(SHY_MODE) -> Terminator4/1
  WOW Module/7(User_Cmd_Out) -> Terminator5/1
  Bus Formatting NG/1(Bus Out) -> WOW Module/3(NG_In)
  Bus Formatting MGL/1(Bus Out) -> WOW Module/4(MGL_In)
  Bus Formatting MGR/1(Bus Out) -> WOW Module/5(MGR_In)
  DSC Load Conversion/1 -> Bus Formatting NG/1(WOW_N)  "Sim.NG_WOW_N"
  DSC Load Conversion/3 -> Bus Formatting MGL/1(WOW_N)  "Sim.MGL_WOW_N"
  DSC Load Conversion/5 -> Bus Formatting MGR/1(WOW_N)  "Sim.MGR_WOW_N"
  Saturation N/1 -> Re-Encoding N/1
  Saturation L/1 -> Re-Encoding L/1
  Saturation R/1 -> Re-Encoding R/1
  Bus Element In1/1 -> Load Cell and Unit Conversion/1(NG Wheel Load Lbf)
  Bus Element In4/1 -> Load Cell and Unit Conversion/2(MGL Wheel Load Lbf)
  Bus Element In5/1 -> Load Cell and Unit Conversion/3(MGR Wheel Load Lbf)
  Load Cell and Unit Conversion/1(NG Cell Load N) -> DSC Data Acquisition/1(NG Cell Load N)
  Load Cell and Unit Conversion/2(MGL Cell Load N) -> DSC Data Acquisition/2(MGL Cell Load N)
  Load Cell and Unit Conversion/3(MGR Cell Load N) -> DSC Data Acquisition/3(MGR Cell Load N)
  DSC Data Acquisition/1(NG DSC Load N) -> Delay3/1
  DSC Data Acquisition/2(MGL DSC Load N) -> Delay1/1
  DSC Data Acquisition/3(MGR DSC Load N) -> Delay2/1
  DSC Load Conversion/2 -> Terminator6/1
  DSC Load Conversion/4 -> Terminator7/1
  DSC Load Conversion/6 -> Terminator8/1

== system Lib_Piccolo/Piccolo State Machine/Landing State Machine/FlareLatch/Latch ==
  D : Inport
  Enable/!Rst : Inport  Port=2
  AND : Logic  IconShape=distinctive  AllPortsSameDT=off  OutDataTypeStr=boolean
  Constant : Constant
  OR : Logic  Operator=OR  IconShape=distinctive  AllPortsSameDT=off  OutDataTypeStr=boolean
  Switch : Switch  Criteria=u2 > Threshold  Threshold=0.5
  Unit Delay : UnitDelay  SampleTime=-1
  Q_Latched : Outport
  wires:
  Unit Delay/1 -> OR/2
  Switch/1 -> Q_Latched/1, Unit Delay/1
  D/1 -> Switch/3, OR/1
  OR/1 -> AND/1
  AND/1 -> Switch/2
  Enable/!Rst/1 -> AND/2
  Constant/1 -> Switch/1

== system Lib_Piccolo/Pitch to Elevator/Reference Frame Conversion and Pitch Rate Limit Determination/AeroVsStruct_Limit/Flap Compensation ==
  CL_Limit_in : Inport
  Gain : Gain  Gain=dCl_per_dFlap
  Sum : Sum  Inputs=|++
  CL_Limit_adjusted : Outport
  wires:
  [flapCmd] -> Gain/1
  Gain/1 -> Sum/2
  Sum/1 -> CL_Limit_adjusted/1
  CL_Limit_in/1 -> Sum/1

== system Lib_Piccolo/WOW Archive Container/Load Cell WoW Model 10/Subsystem/LPF L ==
  Input : Inport
  Reset : Inport  Port=2
  Add1 : Sum  Inputs=++|
  Compare To Constant2 : simulink/Logic and Bit Operations/Compare To Constant  relop=>  const=0  OutDataTypeStr=uint8
  Constant11 : Constant  Value=Cutoff
  Switch1 : Switch  Criteria=u2 > Threshold
  Unit Delay1 : UnitDelay  InitialCondition=Init  SampleTime=-1
  a1 : Gain  Gain=SensorModel.WOW.Cell.a1
  b0 : Gain  Gain=SensorModel.WOW.Cell.b0
  Output : Outport
  wires:
  Unit Delay1/1 -> a1/1
  b0/1 -> Add1/2
  Add1/1 -> Unit Delay1/1, Switch1/1
  a1/1 -> Add1/1
  Input/1 -> Switch1/3, b0/1
  Switch1/1 -> Output/1
  Compare To Constant2/1 -> Switch1/2
  Constant11/1 -> Compare To Constant2/1

== system Lib_Piccolo/WOW Archive Container/Load Cell WoW Model 10/Subsystem/LPF N ==
  Input : Inport
  Reset : Inport  Port=2
  Add1 : Sum  Inputs=++|
  Compare To Constant2 : simulink/Logic and Bit Operations/Compare To Constant  relop=>  const=0  OutDataTypeStr=uint8
  Constant11 : Constant  Value=Cutoff
  Switch1 : Switch  Criteria=u2 > Threshold
  Unit Delay1 : UnitDelay  InitialCondition=Init  SampleTime=-1
  a1 : Gain  Gain=SensorModel.WOW.Cell.a1
  b0 : Gain  Gain=SensorModel.WOW.Cell.b0
  Output : Outport
  wires:
  Unit Delay1/1 -> a1/1
  b0/1 -> Add1/2
  Add1/1 -> Unit Delay1/1, Switch1/1
  a1/1 -> Add1/1
  Input/1 -> Switch1/3, b0/1
  Switch1/1 -> Output/1
  Compare To Constant2/1 -> Switch1/2
  Constant11/1 -> Compare To Constant2/1

== system Lib_Piccolo/WOW Archive Container/Load Cell WoW Model 10/Subsystem/LPF R ==
  Input : Inport
  Reset : Inport  Port=2
  Add1 : Sum  Inputs=++|
  Compare To Constant2 : simulink/Logic and Bit Operations/Compare To Constant  relop=>  const=0  OutDataTypeStr=uint8
  Constant11 : Constant  Value=Cutoff
  Switch1 : Switch  Criteria=u2 > Threshold
  Unit Delay1 : UnitDelay  InitialCondition=Init  SampleTime=-1
  a1 : Gain  Gain=SensorModel.WOW.Cell.a1
  b0 : Gain  Gain=SensorModel.WOW.Cell.b0
  Output : Outport
  wires:
  Unit Delay1/1 -> a1/1
  b0/1 -> Add1/2
  Add1/1 -> Unit Delay1/1, Switch1/1
  a1/1 -> Add1/1
  Input/1 -> Switch1/3, b0/1
  Switch1/1 -> Output/1
  Compare To Constant2/1 -> Switch1/2
  Constant11/1 -> Compare To Constant2/1

== system Lib_Piccolo/WOW Archive Container/Load Cell WoW Model 10/Subsystem/Landing Configuration ==
  Sim.WOW_Filt : Inport
  1-Wheel Timeout : Subsystem  mask{period=SensorModel.WOW.Cell.timeout}
      mask prompts: period "Period [s]"
  AND : Logic  IconShape=distinctive  AllPortsSameDT=off  OutDataTypeStr=boolean
  AND1 : Logic  Inputs=3  IconShape=distinctive  AllPortsSameDT=off  OutDataTypeStr=boolean
  AND2 : Logic  IconShape=distinctive  AllPortsSameDT=off  OutDataTypeStr=boolean
  AND3 : Logic  IconShape=distinctive  AllPortsSameDT=off  OutDataTypeStr=boolean
  Bus Selector : BusSelector  OutputSignals=Sim:WOW_Filt_NG,Sim:WOW_Filt_L,Sim:WOW_Filt_R
  Bus Selector1 : BusSelector  OutputSignals=Sim:WOW_L_N,Sim:WOW_R_N
  Compare To Constant1 : simulink/Logic and Bit Operations/Compare To Constant  relop=>  const=SensorModel.WOW.Cell.loadThresholdUpper3_N  OutDataTypeStr=uint8
  Compare To Constant4 : simulink/Logic and Bit Operations/Compare To Constant  relop=>  const=SensorModel.WOW.Cell.loadThresholdUpper3_N  OutDataTypeStr=uint8
  Constant : Constant  Value=0  OutDataTypeStr=boolean
  Enable : Constant  Value=SensorModel.WOW.Cell.useDualLogic
  Gain1 : Gain
  Gain2 : Gain
  Hysteresis L : Relay  OnSwitchValue=SensorModel.WOW.Cell.loadThresholdUpper_N  OffSwitchValue=SensorModel.WOW.Cell.loadThresholdLower_N
  Hysteresis R : Relay  OnSwitchValue=SensorModel.WOW.Cell.loadThresholdUpper_N  OffSwitchValue=SensorModel.WOW.Cell.loadThresholdLower_N
  Latch : Subsystem
  Latch1 : Subsystem
  NOT : Logic  Operator=NOT  IconShape=distinctive  AllPortsSameDT=off  OutDataTypeStr=boolean
  NOT1 : Logic  Operator=NOT  IconShape=distinctive  AllPortsSameDT=off  OutDataTypeStr=boolean
  NOT2 : Logic  Operator=NOT  IconShape=distinctive  AllPortsSameDT=off  OutDataTypeStr=boolean
  OR : Logic  Operator=OR  IconShape=distinctive  AllPortsSameDT=off  OutDataTypeStr=boolean
  OR1 : Logic  Operator=OR  IconShape=distinctive  AllPortsSameDT=off  OutDataTypeStr=boolean
  Persistance Timer : Subsystem  mask{period=SensorModel.WOW.Cell.persistanceTime_s}
      mask prompts: period "Period [s]"
  Persistance Timer 2 : Subsystem  mask{period=SensorModel.WOW.Cell.persistanceTime2_s}
      mask prompts: period "Period [s]"
  Primary Latch Timer : Subsystem  mask{period=SensorModel.WOW.Cell.longLatchTime_s}
      mask prompts: period "Period [s]"
  Switch : Switch  Criteria=u2 > Threshold  Threshold=0.5
  Switch1 : Switch  Criteria=u2 > Threshold  Threshold=0.5
  Switch2 : Switch  Criteria=u2 > Threshold
  Terminator : Terminator
  Terminator1 : Terminator
  Terminator2 : Terminator
  Unit Delay : UnitDelay  SampleTime=-1
  Unit Delay1 : UnitDelay  SampleTime=-1
  XOR : Logic  Operator=XOR  IconShape=distinctive  AllPortsSameDT=off  OutDataTypeStr=boolean
  ContactBool : Outport
  wires:
  AND3/1 -> 1-Wheel Timeout/1(Enable/!Rst)
  NOT1/1 -> AND2/2
  Primary Latch Timer/1(Expired) -> NOT1/1
  Unit Delay1/1 -> Primary Latch Timer/1(Enable/!Rst)
  Unit Delay/1 -> [Contact]
  [WOWtimeout] -> Switch1/2
  Constant/1 -> Switch1/3
  [WOWtimeout] -> AND2/1
  Switch1/1 -> ContactBool/1
  AND2/1 -> Latch/2(Enable/!Rst)
  NOT/1 -> [WOWtimeout]  "Sim.WOWtimeout"
  1-Wheel Timeout/1(Expired) -> NOT/1
  XOR/1 -> AND3/1
  Enable/1 -> AND1/1
  AND1/1 -> Switch/2, AND3/2  "Logic Mode (And/!Or)"
  [Contact] -> AND1/2
  Switch/1 -> Persistance Timer/1(Enable/!Rst)  "2WheelContact"
  OR/1 -> Switch/1
  Bus Selector/3 -> Hysteresis R/1  "<Sim:WOW_Filt_R>"
  Bus Selector/2 -> Hysteresis L/1  "<Sim:WOW_Filt_L>"
  Bus Selector/1 -> Terminator/1  "<Sim:WOW_Filt_NG>"
  Sim.WOW_Filt/1 -> Bus Selector1/1, Bus Selector/1
  Gain2/1 -> Terminator2/1  "ContactR"
  AND/1 -> Switch/3
  Gain1/1 -> Terminator1/1  "ContactL"
  Hysteresis R/1 -> XOR/2, Gain2/1, AND/2, OR/2
  Hysteresis L/1 -> XOR/1, Gain1/1, AND/1, OR/1
  Persistance Timer/1(Expired) -> Latch/1(D), Switch2/3  "2WheelContactPersistance"
  Bus Selector1/1 -> Compare To Constant4/1  "<Sim:WOW_L_N>"
  Bus Selector1/2 -> Compare To Constant1/1  "<Sim:WOW_R_N>"
  Compare To Constant4/1 -> OR1/1
  Compare To Constant1/1 -> OR1/2
  NOT2/1 -> Switch2/2, AND1/3
  Latch1/1(Q_Latched) -> NOT2/1  "OverLoadLogicLatch"
  Latch/1(Q_Latched) -> Switch2/1, Unit Delay1/1  "ContactBoolLatch"
  Switch2/1 -> Unit Delay/1, Switch1/1  "ContactBool"
  [Contact] -> Latch1/2(Enable/!Rst)
  OR1/1 -> Persistance Timer 2/1(Enable/!Rst)
  Persistance Timer 2/1(Expired) -> Latch1/1(D)

== system Lib_Piccolo/WOW Archive Container/Load Cell WoW Model 10/Subsystem/T//O Configuration ==
  note: Unlike when landing our persistance and latching is inverted relative to Weight Off both gears.
      |
      | Protection against WOW Failure. In the Event of a Sensor Failure and AC lift's off, NZ threshold overides WOW signal.
  Sim.WOW_Filt : Inport
  AND : Logic  IconShape=distinctive  AllPortsSameDT=off  OutDataTypeStr=boolean
  Bus Selector : BusSelector  OutputSignals=Sim:WOW_Filt_NG,Sim:WOW_Filt_L,Sim:WOW_Filt_R
  Compare To Constant1 : simulink/Logic and Bit Operations/Compare To Constant  relop=<  const=SensorModel.WOW.Cell.TO_loadThreshold_N  OutDataTypeStr=uint8
  Compare To Constant2 : simulink/Logic and Bit Operations/Compare To Constant  relop=<  const=SensorModel.WOW.Cell.TO_loadThreshold_N  OutDataTypeStr=uint8
  Latch : Subsystem
  Latch Timer : Subsystem  mask{period=SensorModel.WOW.Cell.TO_latchTime_s}
      mask prompts: period "Period [s]"
  NOT : Logic  Operator=NOT  IconShape=distinctive  AllPortsSameDT=off  OutDataTypeStr=boolean
  NOT2 : Logic  Operator=NOT  IconShape=distinctive  AllPortsSameDT=off  OutDataTypeStr=boolean
  Persistance Timer : Subsystem  mask{period=SensorModel.WOW.Cell.TO_persistanceTime_s}
      mask prompts: period "Period [s]"
  Terminator : Terminator
  Unit Delay : UnitDelay  SampleTime=-1
  ContactBool : Outport
  wires:
  NOT2/1 -> ContactBool/1
  Persistance Timer/1(Expired) -> Latch/1(D)
  Compare To Constant2/1 -> AND/1
  Latch Timer/1(Expired) -> NOT/1
  Unit Delay/1 -> Latch Timer/1(Enable/!Rst)
  Compare To Constant1/1 -> AND/2
  AND/1 -> Persistance Timer/1(Enable/!Rst)
  Latch/1(Q_Latched) -> Unit Delay/1, NOT2/1  "ContactBool"
  NOT/1 -> Latch/2(Enable/!Rst)
  Sim.WOW_Filt/1 -> Bus Selector/1
  Bus Selector/1 -> Terminator/1  "<Sim:WOW_Filt_NG>"
  Bus Selector/2 -> Compare To Constant2/1  "<Sim:WOW_Filt_L>"
  Bus Selector/3 -> Compare To Constant1/1  "<Sim:WOW_Filt_R>"

== system Lib_Piccolo/WOW Archive Container/Load Cell WoW Model 10_OLD/Subsystem/LPF L ==
  Input : Inport
  Reset : Inport  Port=2
  Add1 : Sum  Inputs=++|
  Compare To Constant2 : simulink/Logic and Bit Operations/Compare To Constant  relop=>  const=0  OutDataTypeStr=uint8
  Constant11 : Constant  Value=Cutoff
  Switch1 : Switch  Criteria=u2 > Threshold
  Unit Delay1 : UnitDelay  InitialCondition=Init  SampleTime=-1
  a1 : Gain  Gain=SensorModel.WOW.Cell.a1
  b0 : Gain  Gain=SensorModel.WOW.Cell.b0
  Output : Outport
  wires:
  Constant11/1 -> Compare To Constant2/1
  Compare To Constant2/1 -> Switch1/2
  Switch1/1 -> Output/1
  Input/1 -> b0/1, Switch1/3
  a1/1 -> Add1/1
  Add1/1 -> Switch1/1, Unit Delay1/1
  b0/1 -> Add1/2
  Unit Delay1/1 -> a1/1

== system Lib_Piccolo/WOW Archive Container/Load Cell WoW Model 10_OLD/Subsystem/LPF N ==
  Input : Inport
  Reset : Inport  Port=2
  Add1 : Sum  Inputs=++|
  Compare To Constant2 : simulink/Logic and Bit Operations/Compare To Constant  relop=>  const=0  OutDataTypeStr=uint8
  Constant11 : Constant  Value=Cutoff
  Switch1 : Switch  Criteria=u2 > Threshold
  Unit Delay1 : UnitDelay  InitialCondition=Init  SampleTime=-1
  a1 : Gain  Gain=SensorModel.WOW.Cell.a1
  b0 : Gain  Gain=SensorModel.WOW.Cell.b0
  Output : Outport
  wires:
  Constant11/1 -> Compare To Constant2/1
  Compare To Constant2/1 -> Switch1/2
  Switch1/1 -> Output/1
  Input/1 -> b0/1, Switch1/3
  a1/1 -> Add1/1
  Add1/1 -> Switch1/1, Unit Delay1/1
  b0/1 -> Add1/2
  Unit Delay1/1 -> a1/1

== system Lib_Piccolo/WOW Archive Container/Load Cell WoW Model 10_OLD/Subsystem/LPF R ==
  Input : Inport
  Reset : Inport  Port=2
  Add1 : Sum  Inputs=++|
  Compare To Constant2 : simulink/Logic and Bit Operations/Compare To Constant  relop=>  const=0  OutDataTypeStr=uint8
  Constant11 : Constant  Value=Cutoff
  Switch1 : Switch  Criteria=u2 > Threshold
  Unit Delay1 : UnitDelay  InitialCondition=Init  SampleTime=-1
  a1 : Gain  Gain=SensorModel.WOW.Cell.a1
  b0 : Gain  Gain=SensorModel.WOW.Cell.b0
  Output : Outport
  wires:
  Constant11/1 -> Compare To Constant2/1
  Compare To Constant2/1 -> Switch1/2
  Switch1/1 -> Output/1
  Input/1 -> b0/1, Switch1/3
  a1/1 -> Add1/1
  Add1/1 -> Switch1/1, Unit Delay1/1
  b0/1 -> Add1/2
  Unit Delay1/1 -> a1/1
